simulink model "cmuauv_controller"  (R2026b)
settings: Solver=ode45  StopTime=60
values from neighbouring files (symbols this model uses):
  B = 119.071    [init_cmu_auv.m]    (also in init_cmu_auv_BACKUP_before_casegains.m; init_cmu_auv_BACKUP_before_cases.m = 117.2295; init_cmu_auv_BACKUP_before_ff.m = 117.2295; init_cmu_auv_BACKUP_before_noise.m)
  D_L = [  0,        0,       -5.39181,  0,       -0.02484,  0 ... (first row only)    [init_cmu_auv.m]    (also in init_cmu_auv_BACKUP_before_casegains.m; init_cmu_auv_BACKUP_before_cases.m; init_cmu_auv_BACKUP_before_ff.m; init_cmu_auv_BACKUP_before_noise.m)
  D_Q = [ 55.5498,    0,        1.30135,  0,       -1.17923,  0 ... (first row only)    [init_cmu_auv.m]    (also in init_cmu_auv_BACKUP_before_casegains.m = [  1.30135,   0,        55.54980,  0,       -1.17923,  0; init_cmu_auv_BACKUP_before_cases.m = [  1.30135,   0,        55.54980,  0,       -1.17923,  0; init_cmu_auv_BACKUP_before_ff.m = [  1.30135,   0,        55.54980,  0,       -1.17923,  0; init_cmu_auv_BACKUP_before_noise.m = [  1.30135,   0,        55.54980,  0,       -1.17923,  0)
  dt = 0.05    [init_cmu_auv.m]    (also in init_cmu_auv_BACKUP_before_casegains.m; init_cmu_auv_BACKUP_before_cases.m; init_cmu_auv_BACKUP_before_ff.m; init_cmu_auv_BACKUP_before_noise.m)
  M_total = M_RB + M_A    [init_cmu_auv.m]    (also in init_cmu_auv_BACKUP_before_casegains.m; init_cmu_auv_BACKUP_before_cases.m; init_cmu_auv_BACKUP_before_ff.m; init_cmu_auv_BACKUP_before_noise.m)
  Q_ekf = diag([ones(1,6)*1e-4, ones(1,6)*1e-2])    [init_cmu_auv.m]    (also in init_cmu_auv_BACKUP_before_casegains.m; init_cmu_auv_BACKUP_before_cases.m; init_cmu_auv_BACKUP_before_ff.m; init_cmu_auv_BACKUP_before_noise.m)
  Q_tab = [ ... (first row only)    [init_cmu_auv.m]
  R_ekf = diag([sigma_eta.^2, sigma_gyro.^2])    [init_cmu_auv.m]    (also in init_cmu_auv_BACKUP_before_casegains.m; init_cmu_auv_BACKUP_before_cases.m = diag([1e-2, 1e-2, 1e-3, 1e-3, 1e-3, 1e-3, 1e-2, 1e-2, 1e-2]); init_cmu_auv_BACKUP_before_ff.m = diag([1e-2, 1e-2, 1e-3, 1e-3, 1e-3, 1e-3, 1e-2, 1e-2, 1e-2]); init_cmu_auv_BACKUP_before_noise.m = diag([1e-2, 1e-2, 1e-3, 1e-3, 1e-3, 1e-3, 1e-2, 1e-2, 1e-2]))
  R_tab = [ ... (first row only)    [init_cmu_auv.m]
  sigma_eta = [0.03 0.03 0.01  0.01 0.01 0.01]    [init_cmu_auv.m]    (also in init_cmu_auv_BACKUP_before_casegains.m)
  sigma_gyro = [0.01 0.01 0.01]    [init_cmu_auv.m]    (also in init_cmu_auv_BACKUP_before_casegains.m)
  T_max = 2.7*9.81    (= 26.487)    [init_cmu_auv.m]    (also in init_cmu_auv_BACKUP_before_casegains.m; init_cmu_auv_BACKUP_before_cases.m; init_cmu_auv_BACKUP_before_ff.m; init_cmu_auv_BACKUP_before_noise.m)
  T_min = -2.4*9.81    (= -23.544)    [init_cmu_auv.m]    (also in init_cmu_auv_BACKUP_before_casegains.m; init_cmu_auv_BACKUP_before_cases.m; init_cmu_auv_BACKUP_before_ff.m; init_cmu_auv_BACKUP_before_noise.m)
  TCM = [  0.70711,  0.70711, -0.70711, -0.70711,  0.00000,  0.00000,  0.00000,  0.00000 ... (first row only)    [init_cmu_auv.m]    (also in init_cmu_auv_BACKUP_before_casegains.m; init_cmu_auv_BACKUP_before_cases.m; init_cmu_auv_BACKUP_before_ff.m; init_cmu_auv_BACKUP_before_noise.m)
  TCM_pinv = pinv(TCM)    [init_cmu_auv.m]    (also in init_cmu_auv_BACKUP_before_casegains.m; init_cmu_auv_BACKUP_before_cases.m; init_cmu_auv_BACKUP_before_ff.m; init_cmu_auv_BACKUP_before_noise.m)
undefined symbols (not defined in the file or in its folder): TrajCase
libraries: simulink x2
settings Model: Creator=coachwsk  LastModifiedBy=coachwsk

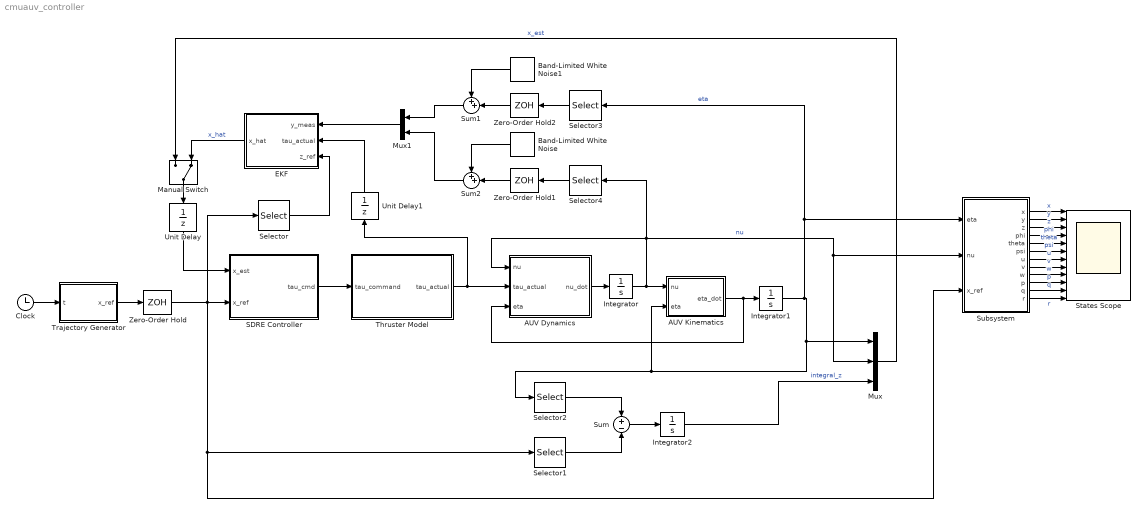
== system cmuauv_controller ==
  AUV Dynamics : MATLAB Function  TreatAsAtomicUnit=on
  AUV Kinematics : MATLAB Function  TreatAsAtomicUnit=on
  Band-Limited White Noise : simulink/Sources/Band-Limited White Noise  Cov=(sigma_gyro.^2)*dt  Ts=0.05  seed=[54321]
  Band-Limited White Noise1 : simulink/Sources/Band-Limited White Noise  Cov=(sigma_eta.^2)*dt  Ts=0.05  seed=[23341]
  Clock : Clock
  EKF : MATLAB Function  TreatAsAtomicUnit=on
  Integrator : Integrator
  Integrator1 : Integrator
  Integrator2 : Integrator  LimitOutput=on  UpperSaturationLimit=10  LowerSaturationLimit=-10
  Manual Switch : ManualSwitch  CurrentSetting=0
  Mux : Mux  Inputs=3
  Mux1 : Mux  Inputs=2
  SDRE Controller : MATLAB Function  TreatAsAtomicUnit=on
  Selector : Selector  InputPortWidth=13  IndexOptions=Index vector (dialog)  Indices=[3]  OutputSizes=1
  Selector1 : Selector  InputPortWidth=13  IndexOptions=Index vector (dialog)  Indices=[3]  OutputSizes=1
  Selector2 : Selector  InputPortWidth=6  IndexOptions=Index vector (dialog)  Indices=[3]  OutputSizes=1
  Selector3 : Selector  InputPortWidth=6  IndexOptions=Index vector (dialog)  Indices=[1 2 3 4 5 6]  OutputSizes=1
  Selector4 : Selector  InputPortWidth=6  IndexOptions=Index vector (dialog)  Indices=[4 5 6]  OutputSizes=1
  States Scope : Scope  NumInputPorts=12
      settings: ActiveDisplayYMinimum=-1.3273704161606072  ActiveDisplayYMaximum=1.9464044181254114
  Subsystem : Subsystem
  Sum : Sum  Inputs=+|-
  Sum1 : Sum  Inputs=++|
  Sum2 : Sum  Inputs=++|
  Thruster Model : Subsystem
  Trajectory Generator : MATLAB Function  TreatAsAtomicUnit=on
  Unit Delay : UnitDelay  SampleTime=-1
  Unit Delay1 : UnitDelay  SampleTime=-1
  Zero-Order Hold : ZeroOrderHold  SampleTime=0.05
  Zero-Order Hold1 : ZeroOrderHold  SampleTime=0.05
  Zero-Order Hold2 : ZeroOrderHold  SampleTime=0.05
  wires:
  Clock/1 -> Trajectory Generator/1(t)
  Trajectory Generator/1(x_ref) -> Zero-Order Hold/1
  Zero-Order Hold/1 -> Selector1/1, Subsystem/3(x_ref), Selector/1, SDRE Controller/2(x_ref)
  EKF/1(x_hat) -> Manual Switch/2  "x_hat"
  Unit Delay/1 -> SDRE Controller/1(x_est)
  Selector/1 -> EKF/3(z_ref)
  Integrator/1 -> Selector4/1, AUV Dynamics/1(nu), Subsystem/2(nu), Mux/2, AUV Kinematics/1(nu)  "nu"
  AUV Dynamics/1(nu_dot) -> Integrator/1
  AUV Kinematics/1(eta_dot) -> AUV Dynamics/3(eta), Integrator1/1
  Integrator1/1 -> Subsystem/1(eta), Selector3/1, Mux/1, AUV Kinematics/2(eta), Selector2/1  "eta"
  SDRE Controller/1(tau_cmd) -> Thruster Model/1(tau_command)
  Thruster Model/1(tau_actual) -> AUV Dynamics/2(tau_actual), Unit Delay1/1
  Unit Delay1/1 -> EKF/2(tau_actual)
  Selector2/1 -> Sum/1
  Selector1/1 -> Sum/2
  Sum/1 -> Integrator2/1
  Integrator2/1 -> Mux/3  "integral_z"
  Selector4/1 -> Zero-Order Hold1/1
  Zero-Order Hold2/1 -> Sum1/2
  Band-Limited White Noise1/1 -> Sum1/1
  Zero-Order Hold1/1 -> Sum2/2
  Band-Limited White Noise/1 -> Sum2/1
  Mux1/1 -> EKF/1(y_meas)
  Sum1/1 -> Mux1/1
  Sum2/1 -> Mux1/2
  Manual Switch/1 -> Unit Delay/1
  Mux/1 -> Manual Switch/1  "x_est"
  Selector3/1 -> Zero-Order Hold2/1
  Subsystem/12(r) -> States Scope/12  "r"
  Subsystem/1(x) -> States Scope/1  "x"
  Subsystem/2(y) -> States Scope/2  "y"
  Subsystem/3(z) -> States Scope/3  "z"
  Subsystem/4(phi) -> States Scope/4  "phi"
  Subsystem/5(theta) -> States Scope/5  "theta"
  Subsystem/6(psi) -> States Scope/6  "psi"
  Subsystem/7(u) -> States Scope/7  "u"
  Subsystem/8(v) -> States Scope/8  "v"
  Subsystem/9(w) -> States Scope/9  "w"
  Subsystem/10(p) -> States Scope/10  "p"
  Subsystem/11(q) -> States Scope/11  "q"

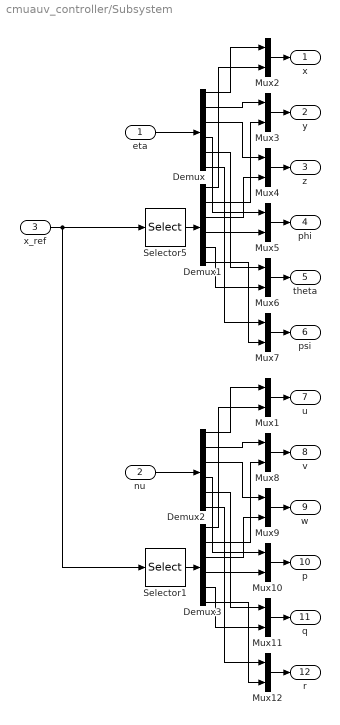
== system cmuauv_controller/Subsystem ==
  eta : Inport
  nu : Inport  Port=2
  x_ref : Inport  Port=3
  Demux{,1..3} (4 alike) : Demux  Outputs=6
  Mux{1..12} (12 alike) : Mux  Inputs=2
  Selector1 : Selector  InputPortWidth=13  IndexOptions=Index vector (dialog)  Indices=[7 8 9 10 11 12]  OutputSizes=1
  Selector5 : Selector  InputPortWidth=13  IndexOptions=Index vector (dialog)  Indices=[1 2 3 4 5 6]  OutputSizes=1
  x : Outport
  y : Outport  Port=2
  z : Outport  Port=3
  phi : Outport  Port=4
  theta : Outport  Port=5
  psi : Outport  Port=6
  u : Outport  Port=7
  v : Outport  Port=8
  w : Outport  Port=9
  p : Outport  Port=10
  q : Outport  Port=11
  r : Outport  Port=12
  wires:
  Mux5/1 -> phi/1
  Mux2/1 -> x/1
  Demux1/6 -> Mux7/2
  Mux6/1 -> theta/1
  Demux1/3 -> Mux4/2
  Mux3/1 -> y/1
  Mux4/1 -> z/1
  Demux1/4 -> Mux5/2
  Demux1/1 -> Mux2/2
  Mux7/1 -> psi/1
  Demux1/5 -> Mux6/2
  Demux/6 -> Mux7/1
  Selector5/1 -> Demux1/1
  x_ref/1 -> Selector1/1, Selector5/1
  Demux/4 -> Mux5/1
  Demux/5 -> Mux6/1
  Demux/3 -> Mux4/1
  Demux1/2 -> Mux3/2
  Demux/2 -> Mux3/1
  Demux/1 -> Mux2/1
  Selector1/1 -> Demux3/1
  Demux2/1 -> Mux1/1
  Mux12/1 -> r/1
  Demux2/2 -> Mux8/1
  Mux9/1 -> w/1
  Mux1/1 -> u/1
  Mux8/1 -> v/1
  Demux2/3 -> Mux9/1
  Mux11/1 -> q/1
  Demux2/6 -> Mux12/1
  Demux3/4 -> Mux10/2
  Demux3/5 -> Mux11/2
  Demux3/2 -> Mux8/2
  Demux3/6 -> Mux12/2
  Demux3/1 -> Mux1/2
  Mux10/1 -> p/1
  Demux2/5 -> Mux11/1
  Demux3/3 -> Mux9/2
  Demux2/4 -> Mux10/1
  eta/1 -> Demux/1
  nu/1 -> Demux2/1

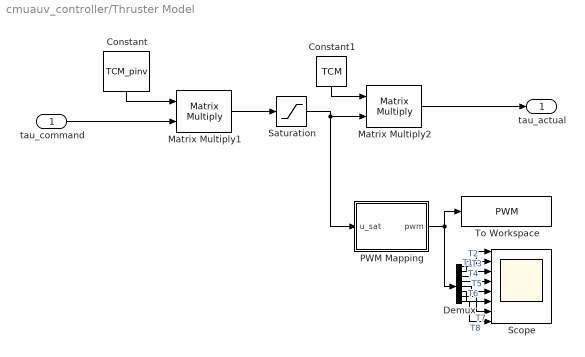
== system cmuauv_controller/Thruster Model ==
  tau_command : Inport
  Constant : Constant  Value=TCM_pinv
  Constant1 : Constant  Value=TCM
  Demux : Demux  Outputs=8
  Matrix Multiply1 : Product  Multiplication=Matrix(*)
  Matrix Multiply2 : Product  Multiplication=Matrix(*)
  PWM Mapping : MATLAB Function  TreatAsAtomicUnit=on
  Saturation : Saturate  UpperLimit=T_max  LowerLimit=T_min
  Scope : Scope  NumInputPorts=8
  To Workspace : ToWorkspace  VariableName=PWM  SaveFormat=Structure With Time  SampleTime=-1
  tau_actual : Outport
  wires:
  Demux/8 -> Scope/8  "T8"
  Matrix Multiply2/1 -> tau_actual/1
  Demux/6 -> Scope/6  "T6"
  Demux/4 -> Scope/4  "T4"
  Demux/2 -> Scope/2  "T2"
  Demux/3 -> Scope/3  "T3"
  Demux/7 -> Scope/7  "T7"
  Demux/5 -> Scope/5  "T5"
  tau_command/1 -> Matrix Multiply1/2
  PWM Mapping/1(pwm) -> To Workspace/1, Demux/1
  Constant/1 -> Matrix Multiply1/1
  Saturation/1 -> PWM Mapping/1(u_sat), Matrix Multiply2/2
  Matrix Multiply1/1 -> Saturation/1
  Demux/1 -> Scope/1  "T1"
  Constant1/1 -> Matrix Multiply2/1

== matlab function cmuauv_controller/SDRE Controller ==
  data: x_est input; tau_cmd output; x_ref input; M_total parameter; D_L parameter; D_Q parameter; Q_tab parameter; R_tab parameter; TrajCase parameter; B parameter
function tau_cmd = fcn(x_est, x_ref, M_total, D_L, D_Q, Q_tab, R_tab, TrajCase, B)
coder.extrinsic('care');

% Pre-allocate extrinsic output (removed the 'info' struct)
P = zeros(13, 13);

% Extract states and force column vectors
x_est = x_est(:);
x_ref = x_ref(:);

eta = x_est(1:6);
nu = x_est(7:12);

% Initialize matrices from workspace parameters
M = M_total;
W = 117.23;   % vehicle weight [N] (Table 3); B (buoyancy) still comes from the workspace
% Per-case LQR weights: column k of Q_tab / R_tab holds the diagonal
% weights tuned for trajectory case k (TrajCase = 1..4).
kc = min(max(round(TrajCase), 1), size(Q_tab, 2));
Q = diag(Q_tab(:, kc));
R = diag(R_tab(:, kc));
zg = 0.0620; zb = 0.0213; xb = 0.0050;

% Compute Error
x_err = x_est - x_ref;

% 1. Kinematic Jacobian J(eta)
phi = eta(4); theta = eta(5); psi = eta(6);
J11 = [cos(psi)*cos(theta), -sin(psi)*cos(phi)+cos(psi)*sin(theta)*sin(phi), sin(psi)*sin(phi)+cos(psi)*cos(phi)*sin(theta);
    sin(psi)*cos(theta), cos(psi)*cos(phi)+sin(phi)*sin(theta)*sin(psi), -cos(psi)*sin(phi)+sin(theta)*sin(psi)*cos(phi);
    -sin(theta),         cos(theta)*sin(phi),                            cos(theta)*cos(phi)];
J22 = [1, sin(phi)*tan(theta), cos(phi)*tan(theta);
    0, cos(phi),           -sin(phi);
    0, sin(phi)/cos(theta), cos(phi)/cos(theta)];
J = [J11, zeros(3,3); zeros(3,3), J22];

% 2. Damping Matrix D(nu)
D_L_safe = abs(diag(diag(D_L)));
D_Q_safe = abs(diag(diag(D_Q)));
D_nu = D_L_safe + D_Q_safe * diag(abs(nu));

% 3. State-Dependent Matrices A(x) and B
A = zeros(13, 13);
A(1:6, 7:12) = J;
A(7:12, 7:12) = -M \ D_nu; 
A(13, 3) = 1; % Integral of depth error

B_mat = zeros(13, 6);
B_mat(7:12, 1:6) = inv(M);

% 4. Compute Non-linear Restoring Forces (Feedforward)
g_eta = [(W-B)*sin(theta);
    -(W-B)*cos(theta)*sin(phi);
    -(W-B)*cos(theta)*cos(phi);
    (zg*W - zb*B)*cos(theta)*sin(phi);
    (zg*W - zb*B)*sin(theta) - (xb*B)*cos(theta)*cos(phi);
    (xb*B)*cos(theta)*sin(phi)];

% 4b. Model-based feedforward of the reference motion (body frame):
%     tau_ff = M*nu_d_dot + C(nu_d)*nu_d + D(nu_d)*nu_d
%     nu_d_dot = backward difference of the velocity reference at the
%     20 Hz control rate (dt_ff must equal the controller sample time).
persistent nu_d_prev
dt_ff = 0.05;
nu_d = x_ref(7:12);
if isempty(nu_d_prev)
    nu_d_prev = nu_d;
end
nu_d_dot = (nu_d - nu_d_prev) / dt_ff;
nu_d_prev = nu_d;
a1d = M(1:3,1:3)*nu_d(1:3) + M(1:3,4:6)*nu_d(4:6);
a2d = M(4:6,1:3)*nu_d(1:3) + M(4:6,4:6)*nu_d(4:6);
S1d = [0, -a1d(3), a1d(2); a1d(3), 0, -a1d(1); -a1d(2), a1d(1), 0];
S2d = [0, -a2d(3), a2d(2); a2d(3), 0, -a2d(1); -a2d(2), a2d(1), 0];
C_d = [zeros(3,3), -S1d; -S1d, -S2d];
D_d = D_L_safe + D_Q_safe * diag(abs(nu_d));
tau_ff = M * nu_d_dot + C_d * nu_d + D_d * nu_d;

% 5. SDRE Solver
persistent K_prev
if isempty(K_prev)
    % Initialize with a safe, empty matrix
    K_prev = zeros(6, 13);
end

% Solve ARE (Request only P to avoid struct class mismatches)
P = care(A, B_mat, Q, R);

% If solution is valid (not empty, NaN, or Inf)
if ~isempty(P) && ~any(isnan(P(:))) && ~any(isinf(P(:)))
    K = R \ (B_mat' * P);
    K_prev = K; % Save as the last known good gain
else
    K = K_prev; % Fallback to previous safe gain
end

% Calculate control law
tau_cmd = -K * x_err + g_eta + tau_ff;

% Final failsafe to prevent Integrator crash
if any(isnan(tau_cmd)) || any(isinf(tau_cmd))
    tau_cmd = zeros(6,1);
end
end

== matlab function cmuauv_controller/Trajectory Generator ==
  data: t input; x_ref output
function x_ref = fcn(t)
% Reference trajectory selector. Cases: 1 station keeping, 2 straight line,
% 3 circle, 4 3D infinity-shape. See cmuauv_trajectory.m for all parameters.
% The case number is read from the base-workspace variable TrajCase.
% x_ref = [x, y, z, phi, theta, psi, u, v, w, p, q, r, int_z]
coder.extrinsic('evalin');
TrajCase = 3;
TrajCase = evalin('base', 'TrajCase');
x_ref = cmuauv_trajectory(t, TrajCase);
end

== matlab function cmuauv_controller/EKF ==
  data: y_meas input; x_hat output; tau_actual input; z_ref input; M_total parameter; D_L parameter; D_Q parameter; Q_ekf parameter; R_ekf parameter
function x_hat = fcn(y_meas, tau_actual, z_ref, M_total, D_L, D_Q, Q_ekf, R_ekf)
    % y_meas: Sensor signals 9x1 [eta(1:6); p; q; r]
    % tau_actual: Control effort 6x1
    y_meas = y_meas(:);
    tau_actual = tau_actual(:);
    
    % Use persistent variables to retain values across time steps
    persistent x_prev P_prev int_z
    if isempty(x_prev)
        x_prev = zeros(12,1); % Initial guess: AUV is stationary
        P_prev = eye(12) * 0.1; 
        int_z = 0;
    end
    
    dt = 0.05; % 20Hz update rate
    M = M_total;
    W = 117.23; B = 119.071; zg = 0.0620; zb = 0.0213; xb = 0.0050;
    
    % ==============================================================
    % 1. PREDICT STEP (Estimate future state using physics model)
    % ==============================================================
    eta = x_prev(1:6);
    nu = x_prev(7:12);
    
    phi = eta(4); theta = eta(5); psi = eta(6);
    cphi = cos(phi); sphi = sin(phi);
    cth  = cos(theta); sth  = sin(theta); tth = tan(theta);
    cpsi = cos(psi); spsi = sin(psi);
    
    % Kinematic Jacobian J(eta)
    J1 = [ cpsi*cth, -spsi*cphi + cpsi*sth*sphi,  spsi*sphi + cpsi*cphi*sth;
           spsi*cth,  cpsi*cphi + sphi*sth*spsi, -cpsi*sphi + sth*spsi*cphi;
          -sth,       cth*sphi,                   cth*cphi ];
    J2 = [ 1, sphi*tth, cphi*tth;
           0, cphi,    -sphi;
           0, sphi/cth, cphi/cth ];
    J = [J1, zeros(3,3); zeros(3,3), J2];
    
    % Calculate Restoring Forces
    g_eta = [(W-B)*sth; -(W-B)*cth*sphi; -(W-B)*cth*cphi;
             (zg*W - zb*B)*cth*sphi; (zg*W - zb*B)*sth - (xb*B)*cth*cphi;
             (xb*B)*cth*sphi];
             
    % Calculate Passive Damping (Matching the plant)
    D_L_safe = abs(diag(diag(D_L)));
    D_Q_safe = abs(diag(diag(D_Q)));
    D_nu = D_L_safe + D_Q_safe * diag(abs(nu));
    
    % Calculate Coriolis (For accurate velocity prediction)
    nu1 = nu(1:3); nu2 = nu(4:6);
    a1 = M(1:3,1:3)*nu1 + M(1:3,4:6)*nu2;
    a2 = M(4:6,1:3)*nu1 + M(4:6,4:6)*nu2;
    S_a1 = [0, -a1(3), a1(2); a1(3), 0, -a1(1); -a1(2), a1(1), 0];
    S_a2 = [0, -a2(3), a2(2); a2(3), 0, -a2(1); -a2(2), a2(1), 0];
    C_nu = [zeros(3,3), -S_a1; -S_a1, -S_a2];
    
    % Nonlinear Prediction
    nu_dot = M \ (tau_actual - C_nu*nu - D_nu*nu - g_eta);
    nu_pred = nu + nu_dot * dt;
    eta_pred = eta + (J * nu) * dt;
    x_pred = [eta_pred; nu_pred];
    
    % Linearized State Transition Matrix (F = I + A*dt)
    A = zeros(12, 12);
    A(1:6, 7:12) = J;
    A(7:12, 7:12) = -M \ D_L_safe; % Use D_L_safe as a proxy for the Jacobian to ensure stability
    F = eye(12) + A * dt;
    
    P_pred = F * P_prev * F' + Q_ekf;
    
    % ==============================================================
    % 2. UPDATE STEP (Correct prediction using actual sensor measurements)
    % ==============================================================
    % H matrix extracts the 9 measured states (6 eta and 3 angular velocities)
    H = zeros(9, 12);
    H(1:6, 1:6) = eye(6);       % Extract position and orientation
    H(7:9, 10:12) = eye(3);     % Extract angular velocities
    
    z_pred = H * x_pred;
    innov = y_meas - z_pred;
    
    % Prevent angle wrap-around errors (Wrap angles to -pi to pi)
    innov(4:6) = atan2(sin(innov(4:6)), cos(innov(4:6)));
    
    S = H * P_pred * H' + R_ekf;
    K = (P_pred * H') / S;
    
    % Update State and Covariance
    x_curr = x_pred + K * innov;
    P_curr = (eye(12) - K * H) * P_pred;
    
    % Save values for the next loop
    x_prev = x_curr;
    P_prev = P_curr;
    
    % ==============================================================
    % 3. ASSEMBLE OUTPUT (Append the 13th state)
    % ==============================================================
    int_z = int_z + (x_curr(3) - z_ref) * dt;
    
    x_hat = [x_curr; int_z];
end

== matlab function cmuauv_controller/AUV Dynamics ==
  data: nu_dot output; nu input; tau_actual input; eta input; M_total parameter; D_Q parameter; D_L parameter
function nu_dot = fcn(nu, tau_actual, eta, M_total, D_Q, D_L)
% Force column vectors
tau_actual = tau_actual(:);
nu = nu(:);
eta = eta(:);

M = M_total;
W = 117.23; B = 119.071; zg = 0.0620; zb = 0.0213; xb = 0.0050;

phi = eta(4); theta = eta(5);
g_eta = [(W-B)*sin(theta); 
    -(W-B)*cos(theta)*sin(phi); 
    -(W-B)*cos(theta)*cos(phi);
    (zg*W - zb*B)*cos(theta)*sin(phi); 
    (zg*W - zb*B)*sin(theta) - (xb*B)*cos(theta)*cos(phi);
    (xb*B)*cos(theta)*sin(phi)];

D_L_safe = abs(diag(diag(D_L)));
D_Q_safe = abs(diag(diag(D_Q)));
D_nu = D_L_safe + D_Q_safe * diag(abs(nu));

% =========================================================
% Fossen's Coriolis and Centripetal Matrix C(nu)
% =========================================================
% 1. Split velocities into linear (nu1) and angular (nu2)
nu1 = nu(1:3);
nu2 = nu(4:6);

% 2. Split Total Mass Matrix into 3x3 sub-matrices
M11 = M(1:3, 1:3);
M12 = M(1:3, 4:6);
M21 = M(4:6, 1:3);
M22 = M(4:6, 4:6);

% 3. Calculate terms for the skew-symmetric operator
a1 = M11 * nu1 + M12 * nu2;
a2 = M21 * nu1 + M22 * nu2;

% 4. Explicit Skew-symmetric matrices S(a1) and S(a2)
S_a1 = [   0,   -a1(3),  a1(2); 
    a1(3),    0,   -a1(1); 
    -a1(2),  a1(1),    0   ];

S_a2 = [   0,   -a2(3),  a2(2); 
    a2(3),    0,   -a2(1); 
    -a2(2),  a2(1),    0   ];

% 5. Assemble the full 6x6 C(nu) matrix
C_nu = [ zeros(3,3),  -S_a1;
    -S_a1,     -S_a2 ];
% =========================================================

% Full Nonlinear 6-DOF Equations of Motion
nu_dot = M \ (tau_actual - C_nu * nu - D_nu * nu - g_eta);
end

== matlab function cmuauv_controller/Thruster Model/PWM Mapping ==
  data: u_sat input; pwm output
function pwm = fcn(u_sat)
% Convert bounded thrust (Newtons) to PWM signal (1000 - 2000 us)
pwm = zeros(8,1);

% Max thrust in Surge(forward) requires specific ESC wiring logic:
% T1, T2, T5, T6 = 1000 | T3, T4 = 2000
% Assuming standard base mapping where 1500 is stop, we invert specific channels 
% to match the hardware wiring configuration for the APISQUEEN thrusters.

for i = 1:8
    % Generic linear interpolation (replace with your exact thrust curve)
    if u_sat(i) > 0
        base_pwm = 1500 + (u_sat(i) / 26.487) * 500; 
    else
        base_pwm = 1500 + (u_sat(i) / 23.544) * 500; 
    end

    % Apply hardware-specific inversions to match your Surge wiring example
    if i == 1 || i == 2 || i == 5 || i == 6
        pwm(i) = 3000 - base_pwm; % Inverts so positive thrust yields 1000
    else
        pwm(i) = base_pwm; % Positive thrust yields 2000
    end
end
end

== matlab function cmuauv_controller/AUV Kinematics ==
  data: nu input; eta_dot output; eta input
function eta_dot = fcn(nu, eta)
% Extract Euler angles (roll, pitch, yaw)
phi = eta(4);
theta = eta(5);
psi = eta(6);

% Precompute trigonometric functions to save calculation time
cphi = cos(phi); sphi = sin(phi);
cth  = cos(theta); sth  = sin(theta); tth = tan(theta);
cpsi = cos(psi); spsi = sin(psi);

% J1: Linear velocity transformation matrix (Body to Earth)
J1 = [ cpsi*cth, -spsi*cphi + cpsi*sth*sphi,  spsi*sphi + cpsi*cphi*sth;
    spsi*cth,  cpsi*cphi + sphi*sth*spsi, -cpsi*sphi + sth*spsi*cphi;
    -sth,       cth*sphi,                   cth*cphi ];

% J2: Angular velocity transformation matrix (Body to Earth)
% Note: A kinematic singularity exists at pitch (theta) = +/- 90 degrees.
J2 = [ 1, sphi*tth, cphi*tth;
    0, cphi,    -sphi;
    0, sphi/cth, cphi/cth ];

% Assemble the full 6x6 Jacobian matrix
J = [J1, zeros(3,3);
    zeros(3,3), J2];

% Compute the derivative of the earth-fixed states
eta_dot = J * nu;
end
